simulink model "BoostPFC_Design_VoltageQualified"  (R2024b)
settings: Solver=FixedStepDiscrete  StartTime=0  StopTime=sim_stop_time  FixedStep=Ts_sim  RelTol=1e-3
InitFcn:
  | modelFile = get_param(bdroot, 'FileName'); run(fullfile(fileparts(modelFile), 'BoostPFC_Design_VoltageQualified_Init.m')); clear modelFile
values from neighbouring files (symbols this model uses):
  C_out = 2200e-6    (= 0.0022)    [BoostPFC_Design_Init.m]
  duty_max = 0.95    [BoostPFC_Design_Init.m]
  duty_min = 0.0    (= 0)    [BoostPFC_Design_Init.m]
  f_line = 50    [BoostPFC_Design_Init.m]
  f_sw = 50e3    (= 50000)    [BoostPFC_Design_Init.m]
  Ipk_limit = 4.5    [BoostPFC_Design_Init.m]
  Ki_i = Kp_i*2*pi*fz_i    (= 695.807110277)    [BoostPFC_Design_Init.m]
  Ki_v = Kp_v*2*pi*fz_v    [BoostPFC_Design_Init.m]
  Kp_i = 2*pi*fc_i_target*L_boost/Vout_ref    (= 0.221482282078)    [BoostPFC_Design_Init.m]
  Kp_v = 2*pi*fc_v_target/gvi_coefficient    [BoostPFC_Design_Init.m]
  L_boost = 470e-6    (= 0.00047)    [BoostPFC_Design_Init.m]
  load_step_mode = 0    [BoostPFC_Design_Init.m]    (also in Run_BoostPFC_Design_Cases.m = stepModes(caseIndex))
  load_step_time = 0.45    [BoostPFC_Design_Init.m]    (also in Run_BoostPFC_Design_Cases.m = 0.7)
  precharge_qualification_time = 5e-3    (= 0.005)    [BoostPFC_Design_VoltageQualified_Init.m]
  precharge_resistance = 10    [BoostPFC_Design_Init.m]
  precharge_timeout_time = 0.50    (= 0.5)    [BoostPFC_Design_VoltageQualified_Init.m]
  precharge_voltage_threshold = precharge_voltage_fraction*precharge_passive_ceiling_V    [BoostPFC_Design_VoltageQualified_Init.m]
  Rds_on_effective = Rds_on    (= 0.04)    [BoostPFC_Design_Init.m]    (also in Run_Ideal_Component_Comparison.m = 0)
  rL_effective = rL    (= 0.1)    [BoostPFC_Design_Init.m]    (also in Run_Ideal_Component_Comparison.m = 0)
  Rload_nominal = 40    [BoostPFC_Design_Init.m]
  Rload_precharge = 1e9    (= 1000000000)    [BoostPFC_Design_Init.m]
  softstart_time = 0.25    [BoostPFC_Design_Init.m]
  Ts_sim = 1 / (20 * f_sw)    (= 1e-06)    [BoostPFC_Design_Init.m]
  Vac_rms = 24    [BoostPFC_Design_Init.m]    (also in Run_BoostPFC_Design_Cases.m)
  Vf_boost_effective = Vf_boost    (= 0.65)    [BoostPFC_Design_Init.m]    (also in Run_Ideal_Component_Comparison.m = 0)
  Vf_bridge_effective = Vf_bridge    (= 0.7)    [BoostPFC_Design_Init.m]    (also in Run_Ideal_Component_Comparison.m = 0)
  Vout_ref = 40    [BoostPFC_Design_Init.m]
settings Model: Creator=86133  LastModifiedBy=86133
settings DataIOCC: SaveOutput=off  SaveTime=off

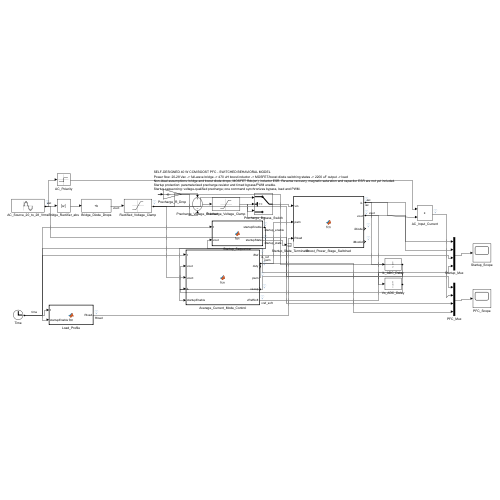
[thumbnail: Simulink's stored preview of the top-level diagram]
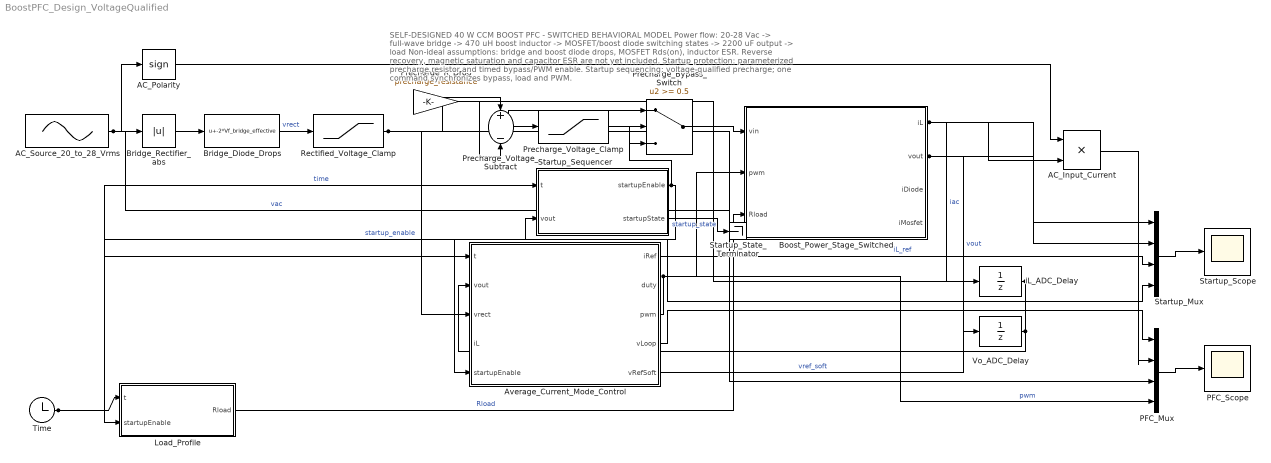
== system BoostPFC_Design_VoltageQualified ==
  note: SELF-DESIGNED 40 W CCM BOOST PFC - SWITCHED BEHAVIORAL MODEL
      | Power flow: 20-28 Vac -> full-wave bridge -> 470 uH boost inductor -> MOSFET/boost diode switching states -> 2200 uF output -> load
      | Non-ideal assumptions: bridge and boost diode drops, MOSFET Rds(on), inductor ESR. Reverse recovery, magnetic saturation and capacitor ESR are not yet included.
      | Startup protection: parameterized precharge resistor and timed bypass/PWM enable.
      | Startup sequencing: voltage-qualified precharge; one command synchronizes bypass, load and PWM.
  AC_Input_Current : Product
  AC_Polarity : Signum
  AC_Source_20_to_28_Vrms : Sin  Amplitude=sqrt(2)*Vac_rms  Frequency=2*pi*f_line  SampleTime=Ts_sim
  Average_Current_Mode_Control : MATLAB Function  TreatAsAtomicUnit=on
  Boost_Power_Stage_Switched : MATLAB Function  TreatAsAtomicUnit=on
  Bridge_Diode_Drops : Bias  Bias=-2*Vf_bridge_effective  SaturateOnIntegerOverflow=off
  Bridge_Rectifier_abs : Abs  SaturateOnIntegerOverflow=off
  Load_Profile : MATLAB Function  TreatAsAtomicUnit=on
  PFC_Mux : Mux
  PFC_Scope : Scope
  Precharge_Bypass_Switch : Switch  Threshold=0.5  SaturateOnIntegerOverflow=off  InputSameDT=off
  Precharge_R_Drop : Gain  Gain=precharge_resistance
  Precharge_Voltage_Clamp : Saturate  UpperLimit=inf  LowerLimit=0
  Precharge_Voltage_Subtract : Sum  Inputs=+-
  Rectified_Voltage_Clamp : Saturate  UpperLimit=inf  LowerLimit=0
  Startup_Mux : Mux
  Startup_Scope : Scope
  Startup_Sequencer : MATLAB Function  TreatAsAtomicUnit=on
  Startup_State_Terminator : Terminator
  Time : Clock
  Vo_ADC_Delay : UnitDelay  SampleTime=Ts_sim  HasFrameUpgradeWarning=on
  iL_ADC_Delay : UnitDelay  SampleTime=Ts_sim  HasFrameUpgradeWarning=on
  wires:
  AC_Source_20_to_28_Vrms/1 -> Bridge_Rectifier_abs/1, AC_Polarity/1, PFC_Mux/1  "vac"
  Bridge_Rectifier_abs/1 -> Bridge_Diode_Drops/1
  Bridge_Diode_Drops/1 -> Rectified_Voltage_Clamp/1  "vrect"
  Time/1 -> Load_Profile/1(t), Average_Current_Mode_Control/1(t), Startup_Sequencer/1(t)  "time"
  Rectified_Voltage_Clamp/1 -> Average_Current_Mode_Control/3(vrect), PFC_Mux/3, Precharge_Voltage_Subtract/1, Precharge_Bypass_Switch/1
  Average_Current_Mode_Control/3(pwm) -> Boost_Power_Stage_Switched/2(pwm), PFC_Mux/4  "pwm"
  Load_Profile/1(Rload) -> Boost_Power_Stage_Switched/3(Rload)  "Rload"
  Vo_ADC_Delay/1 -> Average_Current_Mode_Control/2(vout), Startup_Sequencer/2(vout)
  iL_ADC_Delay/1 -> Average_Current_Mode_Control/4(iL), Precharge_R_Drop/1
  Boost_Power_Stage_Switched/1(iL) -> iL_ADC_Delay/1, AC_Input_Current/2, Startup_Mux/2  "iac"
  Boost_Power_Stage_Switched/2(vout) -> Vo_ADC_Delay/1, Startup_Mux/1  "vout"
  AC_Polarity/1 -> AC_Input_Current/1
  Average_Current_Mode_Control/1(iRef) -> Startup_Mux/3  "iL_ref"
  Average_Current_Mode_Control/5(vRefSoft) -> Startup_Mux/4  "vref_soft"
  Startup_Mux/1 -> Startup_Scope/1
  AC_Input_Current/1 -> PFC_Mux/2
  PFC_Mux/1 -> PFC_Scope/1
  Precharge_R_Drop/1 -> Precharge_Voltage_Subtract/2
  Precharge_Voltage_Subtract/1 -> Precharge_Voltage_Clamp/1
  Precharge_Voltage_Clamp/1 -> Precharge_Bypass_Switch/3
  Precharge_Bypass_Switch/1 -> Boost_Power_Stage_Switched/1(vin)
  Startup_Sequencer/1(startupEnable) -> Precharge_Bypass_Switch/2, Load_Profile/2(startupEnable), Average_Current_Mode_Control/5(startupEnable)  "startup_enable"
  Startup_Sequencer/2(startupState) -> Startup_State_Terminator/1  "startup_state"

== matlab function BoostPFC_Design_VoltageQualified/Load_Profile ==
  data: t input size=1; Rload output size=1; startupEnable input size=1; load_step_mode parameter size=1; Rload_nominal parameter size=1; load_step_time parameter size=1; Rload_precharge parameter size=1
function Rload = fcn(t,startupEnable, load_step_mode, Rload_nominal, load_step_time, Rload_precharge)
% Load remains open until the startup sequencer qualifies precharge.
if startupEnable < 0.5
    Rload = Rload_precharge;
elseif load_step_mode == 1
    if t < load_step_time, Rload = 2*Rload_nominal; else, Rload = Rload_nominal; end
elseif load_step_mode == 2
    if t < load_step_time, Rload = Rload_nominal; else, Rload = 2*Rload_nominal; end
else
    Rload = Rload_nominal;
end

== matlab function BoostPFC_Design_VoltageQualified/Boost_Power_Stage_Switched ==
  data: vin input size=1; iL output size=1; pwm input size=1; Rload input size=1; vout output size=1; iDiode output size=1; iMosfet output size=1; Ts_sim parameter; L_boost parameter; C_out parameter; rL_effective parameter; Rds_on_effective parameter; Vf_boost_effective parameter
function [iL,vout,iDiode,iMosfet] = fcn(vin,pwm,Rload, Ts_sim, L_boost, C_out, rL_effective, Rds_on_effective, Vf_boost_effective)
% Cycle-resolved switched boost equations.
persistent iState vState
if isempty(iState), iState=0; vState=0; end
loadCurrent=vState/max(Rload,1e-6);
if pwm>=0.5
 di=(vin-iState*(rL_effective+Rds_on_effective))/L_boost; dv=-loadCurrent/C_out; iMosfet=iState; iDiode=0;
else
 if (iState>0)||(vin>vState+Vf_boost_effective)
  di=(vin-vState-Vf_boost_effective-iState*rL_effective)/L_boost; iDiode=max(iState,0); dv=(iDiode-loadCurrent)/C_out;
 else
  di=0; iState=0; iDiode=0; dv=-loadCurrent/C_out;
 end
 iMosfet=0;
end
iState=max(iState+Ts_sim*di,0); vState=max(vState+Ts_sim*dv,0); iL=iState; vout=vState;

== matlab function BoostPFC_Design_VoltageQualified/Startup_Sequencer ==
  data: t input size=1; startupEnable output size=1; vout input size=1; startupState output size=1; Ts_sim parameter size=1; precharge_voltage_threshold parameter size=1; precharge_qualification_time parameter size=1; precharge_timeout_time parameter size=1
function [startupEnable,startupState] = fcn(t,vout, Ts_sim, precharge_voltage_threshold, precharge_qualification_time, precharge_timeout_time)
% 0=precharge, 1=qualified/enabled, -1=timeout safe state.
persistent qualifyDuration latched timedOut
if isempty(qualifyDuration), qualifyDuration=0; latched=false; timedOut=false; end
if ~latched && ~timedOut
    if vout >= precharge_voltage_threshold
        qualifyDuration=qualifyDuration+Ts_sim;
    else
        qualifyDuration=0;
    end
    if qualifyDuration >= precharge_qualification_time
        latched=true;
    elseif t >= precharge_timeout_time
        timedOut=true;
    end
end
startupEnable=double(latched);
if timedOut, startupState=-1; elseif latched, startupState=1; else, startupState=0; end

== matlab function BoostPFC_Design_VoltageQualified/Average_Current_Mode_Control ==
  data: t input size=1; iRef output size=1; vout input size=1; vrect input size=1; iL input size=1; duty output size=1; pwm output size=1; vLoop output size=1; vRefSoft output size=1; startupEnable input size=1; Ts_sim parameter size=1; f_sw parameter size=1; Vout_ref parameter size=1; Vac_rms parameter size=1; Kp_v parameter size=1; Ki_v parameter size=1; Kp_i parameter size=1; Ki_i parameter size=1; Ipk_limit parameter size=1; duty_min parameter size=1; duty_max parameter size=1; softstart_time parameter size=1
function [iRef,duty,pwm,vLoop,vRefSoft] = fcn(t,vout,vrect,iL,startupEnable, Ts_sim, f_sw, Vout_ref, Vac_rms, Kp_v, Ki_v, Kp_i, Ki_i, Ipk_limit, duty_min, duty_max, softstart_time)
% Existing average-current-mode control released by startup sequencer.
persistent intV intI carrier enableTime
if isempty(intV), intV=0; intI=0; carrier=0; enableTime=-1; end
if startupEnable < 0.5
    intV=0; intI=0; carrier=0; enableTime=-1;
    iRef=0; duty=0; pwm=0; vLoop=0; vRefSoft=0; return;
end
if enableTime < 0, enableTime=t; end
controlTime=max(t-enableTime,0);
vRefSoft=Vout_ref*min(controlTime/softstart_time,1);
eV=vRefSoft-vout; vUnsat=Kp_v*eV+intV;
vLoop=min(max(vUnsat,0),Ipk_limit);
if (vUnsat==vLoop)||(vUnsat>Ipk_limit&&eV<0)||(vUnsat<0&&eV>0), intV=intV+Ki_v*Ts_sim*eV; end
vPeak=max(sqrt(2)*Vac_rms,1); iRef=min(Ipk_limit,max(0,vLoop*vrect/vPeak));
eI=iRef-iL; dFeedforward=1-vrect/max(Vout_ref,1); dUnsat=dFeedforward+Kp_i*eI+intI;
duty=min(max(dUnsat,duty_min),duty_max);
if (dUnsat==duty)||(dUnsat>duty_max&&eI<0)||(dUnsat<duty_min&&eI>0), intI=intI+Ki_i*Ts_sim*eI; end
carrier=carrier+f_sw*Ts_sim; if carrier>=1, carrier=carrier-floor(carrier); end
pwm=double(duty>carrier);
